simulink model "rfsoc4x2_ospfb_128"  (R2021a)
settings: Solver=VariableStepAuto  StartTime=0.0  StopTime=2048  RelTol=1e-3
undefined symbols (not defined in the file): pfb_coeff_gen_calc
libraries: xbsIndex_r4 x25898, casper_library_delays x113, casper_library_misc x68, xps_library x1
(part 146 of 221)

== system rfsoc4x2_ospfb_128/fft1/fft_direct/butterfly1_0/twiddle/bus_mult/mult1 ==
  a : Inport
  b : Inport  Port=2
  a_expand : Subsystem  AncestorBlock=casper_library_flow_control/bus_expand  mask(bus_expand){mode=divisions of equal size, outputNum=4, outputWidth=[18 18 18 18], outputBinaryPt=[17 17 17 17], outputArithmeticType=[1 1 1 1], show_format=off, outputToWorkspace=off, variablePrefix=out, outputToModelAsWell=on}
      mask prompts: outputNum "Number of outputs:"; outputWidth "Output width:"; outputBinaryPt "Output binary point position:"; outputArithmeticType "Output arithmetic type (ufix=0, fix=1, bool=2):"; show_format "Print format string?"; outputToWorkspace "Output to workspace?"; variablePrefix "Variable name prefix:"; outputToModelAsWell "Output to model as well?"
      mask help:
      | Expands a 'bus' made using a bus_create or Xilinx
      | concat block.
      | The input will be divided into the specified number
      | of outputs with the specified arithmetic types.
      | Divisions are made from most significant bit.
      mask init: same as rfsoc4x2_ospfb_128/bus_expand
      settings: AttributesFormatString=4 outputs
      mask TypeOptions mode: divisions of equal size | divisions of arbitrary size
      mask Callback mode: %bus_expand_callback();
      mask Callback outputWidth: %bus_expand_callback();
      mask Callback outputToWorkspace: %bus_expand_callback();
  a_replicate : Subsystem  AncestorBlock=casper_library_bus/bus_replicate  mask(bus_replicate){replication=2, csp_latency=0, misc=off, implementation=core}
      mask prompts: replication "replication factor"; csp_latency "latency"; misc "misc support"; implementation "delay implementation"
      mask help: Output bus formed by replicating input bus a number of times
      mask init:
      | bus_replicate_init(gcb, ...
      |     'replication', replication, ...
      |     'csp_latency', csp_latency, ...
      |     'implementation', implementation, ...
      |     'misc', misc);
      mask TypeOptions implementation: core | behavioral
  addsub_im : xbsIndex_r4/AddSub  mode=Addition  use_carryin=off  use_carryout=off  en=off  latency=2  precision=Full  arith_type=Unsigned  n_bits=16  bin_pt=14  quantization=Truncate  overflow=Wrap  use_behavioral_HDL=on  hw_selection=Fabric  pipelined=on  use_rpm=on  dbl_ovrd=off  block_type=addsub
  addsub_re : xbsIndex_r4/AddSub  mode=Subtraction  use_carryin=off  use_carryout=off  en=off  latency=2  precision=Full  arith_type=Unsigned  n_bits=16  bin_pt=14  quantization=Truncate  overflow=Wrap  use_behavioral_HDL=on  hw_selection=Fabric  pipelined=on  use_rpm=on  dbl_ovrd=off  block_type=addsub
  b_expand : Subsystem  AncestorBlock=casper_library_flow_control/bus_expand  mask(bus_expand){mode=divisions of equal size, outputNum=4, outputWidth=[18 18 18 18], outputBinaryPt=[17 17 17 17], outputArithmeticType=[1 1 1 1], show_format=off, outputToWorkspace=off, variablePrefix=out, outputToModelAsWell=on}
      mask prompts: outputNum "Number of outputs:"; outputWidth "Output width:"; outputBinaryPt "Output binary point position:"; outputArithmeticType "Output arithmetic type (ufix=0, fix=1, bool=2):"; show_format "Print format string?"; outputToWorkspace "Output to workspace?"; variablePrefix "Variable name prefix:"; outputToModelAsWell "Output to model as well?"
      mask help:
      | Expands a 'bus' made using a bus_create or Xilinx
      | concat block.
      | The input will be divided into the specified number
      | of outputs with the specified arithmetic types.
      | Divisions are made from most significant bit.
      mask init: same as rfsoc4x2_ospfb_128/bus_expand
      settings: AttributesFormatString=4 outputs
      mask TypeOptions mode: divisions of equal size | divisions of arbitrary size
      mask Callback mode: %bus_expand_callback();
      mask Callback outputWidth: %bus_expand_callback();
      mask Callback outputToWorkspace: %bus_expand_callback();
  b_replicate : Subsystem  AncestorBlock=casper_library_bus/bus_replicate  mask(bus_replicate){replication=2, csp_latency=0, misc=off, implementation=core}
      mask prompts: replication "replication factor"; csp_latency "latency"; misc "misc support"; implementation "delay implementation"
      mask help: Output bus formed by replicating input bus a number of times
      mask init:
      | bus_replicate_init(gcb, ...
      |     'replication', replication, ...
      |     'csp_latency', csp_latency, ...
      |     'implementation', implementation, ...
      |     'misc', misc);
      mask TypeOptions implementation: core | behavioral
  convert_im : xbsIndex_r4/Convert  gui_display_data_type=Fixed-point  arith_type="Signed  (2's comp)"  n_bits=37  bin_pt=34  float_type=Single  exp_bits=8  fraction_bits=24  quantization=Truncate  overflow=Wrap  en=off  latency=0  pipeline=on  dbl_ovrd=off  block_type=convert
  convert_re : xbsIndex_r4/Convert  gui_display_data_type=Fixed-point  arith_type="Signed  (2's comp)"  n_bits=37  bin_pt=34  float_type=Single  exp_bits=8  fraction_bits=24  quantization=Truncate  overflow=Wrap  en=off  latency=0  pipeline=on  dbl_ovrd=off  block_type=convert
  imim : xbsIndex_r4/Mult  precision=Full  arith_type="Signed  (2's comp)"  n_bits=16  bin_pt=14  quantization=Truncate  overflow=Wrap  en=off  latency=2  use_behavioral_HDL=on  opt=Speed  use_embedded=off  optimum_pipeline=off  pipeline=on  dbl_ovrd=off  use_rpm=on  placement_style=Triangular  block_type=mult
  imre : xbsIndex_r4/Mult  precision=Full  arith_type="Signed  (2's comp)"  n_bits=16  bin_pt=14  quantization=Truncate  overflow=Wrap  en=off  latency=2  use_behavioral_HDL=on  opt=Speed  use_embedded=off  optimum_pipeline=off  pipeline=on  dbl_ovrd=off  use_rpm=on  placement_style=Triangular  block_type=mult
  reim : xbsIndex_r4/Mult  precision=Full  arith_type="Signed  (2's comp)"  n_bits=16  bin_pt=14  quantization=Truncate  overflow=Wrap  en=off  latency=2  use_behavioral_HDL=on  opt=Speed  use_embedded=off  optimum_pipeline=off  pipeline=on  dbl_ovrd=off  use_rpm=on  placement_style=Triangular  block_type=mult
  rere : xbsIndex_r4/Mult  precision=Full  arith_type="Signed  (2's comp)"  n_bits=16  bin_pt=14  quantization=Truncate  overflow=Wrap  en=off  latency=2  use_behavioral_HDL=on  opt=Speed  use_embedded=off  optimum_pipeline=off  pipeline=on  dbl_ovrd=off  use_rpm=on  placement_style=Triangular  block_type=mult
  ri_to_c : Subsystem  AncestorBlock=casper_library_misc/ri_to_c  mask(ri_to_c){}
      mask help:
      | Concatenates real and imaginary inputs into a complex output.
      | Useful for simplifying interconnects.
      | See also: Complex to Real-Imag (c_to_ri)
      mask Help: eval('xlWeb(''http://casper.berkeley.edu/wiki/Ri_to_c'')')
  ab : Outport
  wires:
  a/1 -> a_replicate/1(in)
  b/1 -> b_replicate/1(in)
  a_replicate/1(out) -> a_expand/1(bus_in)
  b_replicate/1(out) -> b_expand/1(bus_in)
  a_expand/1(msb_out4) -> rere/1
  b_expand/1(msb_out4) -> rere/2
  a_expand/2(out3) -> imim/1
  b_expand/2(out3) -> imim/2
  a_expand/4(lsb_out1) -> imre/1
  b_expand/3(out2) -> imre/2
  a_expand/3(out2) -> reim/1
  b_expand/4(lsb_out1) -> reim/2
  rere/1 -> addsub_re/1
  imim/1 -> addsub_re/2
  imre/1 -> addsub_im/1
  reim/1 -> addsub_im/2
  addsub_re/1 -> convert_re/1
  addsub_im/1 -> convert_im/1
  convert_re/1 -> ri_to_c/1(re)
  convert_im/1 -> ri_to_c/2(im)
  ri_to_c/1(c) -> ab/1

== system rfsoc4x2_ospfb_128/fft1/fft_direct/butterfly1_0/twiddle/bus_mult/mult2 ==
  a : Inport
  b : Inport  Port=2
  a_expand : Subsystem  AncestorBlock=casper_library_flow_control/bus_expand  mask(bus_expand){mode=divisions of equal size, outputNum=4, outputWidth=[18 18 18 18], outputBinaryPt=[17 17 17 17], outputArithmeticType=[1 1 1 1], show_format=off, outputToWorkspace=off, variablePrefix=out, outputToModelAsWell=on}
      mask prompts: outputNum "Number of outputs:"; outputWidth "Output width:"; outputBinaryPt "Output binary point position:"; outputArithmeticType "Output arithmetic type (ufix=0, fix=1, bool=2):"; show_format "Print format string?"; outputToWorkspace "Output to workspace?"; variablePrefix "Variable name prefix:"; outputToModelAsWell "Output to model as well?"
      mask help:
      | Expands a 'bus' made using a bus_create or Xilinx
      | concat block.
      | The input will be divided into the specified number
      | of outputs with the specified arithmetic types.
      | Divisions are made from most significant bit.
      mask init: same as rfsoc4x2_ospfb_128/bus_expand
      settings: AttributesFormatString=4 outputs
      mask TypeOptions mode: divisions of equal size | divisions of arbitrary size
      mask Callback mode: %bus_expand_callback();
      mask Callback outputWidth: %bus_expand_callback();
      mask Callback outputToWorkspace: %bus_expand_callback();
  a_replicate : Subsystem  AncestorBlock=casper_library_bus/bus_replicate  mask(bus_replicate){replication=2, csp_latency=0, misc=off, implementation=core}
      mask prompts: replication "replication factor"; csp_latency "latency"; misc "misc support"; implementation "delay implementation"
      mask help: Output bus formed by replicating input bus a number of times
      mask init:
      | bus_replicate_init(gcb, ...
      |     'replication', replication, ...
      |     'csp_latency', csp_latency, ...
      |     'implementation', implementation, ...
      |     'misc', misc);
      mask TypeOptions implementation: core | behavioral
  addsub_im : xbsIndex_r4/AddSub  mode=Addition  use_carryin=off  use_carryout=off  en=off  latency=2  precision=Full  arith_type=Unsigned  n_bits=16  bin_pt=14  quantization=Truncate  overflow=Wrap  use_behavioral_HDL=on  hw_selection=Fabric  pipelined=on  use_rpm=on  dbl_ovrd=off  block_type=addsub
  addsub_re : xbsIndex_r4/AddSub  mode=Subtraction  use_carryin=off  use_carryout=off  en=off  latency=2  precision=Full  arith_type=Unsigned  n_bits=16  bin_pt=14  quantization=Truncate  overflow=Wrap  use_behavioral_HDL=on  hw_selection=Fabric  pipelined=on  use_rpm=on  dbl_ovrd=off  block_type=addsub
  b_expand : Subsystem  AncestorBlock=casper_library_flow_control/bus_expand  mask(bus_expand){mode=divisions of equal size, outputNum=4, outputWidth=[18 18 18 18], outputBinaryPt=[17 17 17 17], outputArithmeticType=[1 1 1 1], show_format=off, outputToWorkspace=off, variablePrefix=out, outputToModelAsWell=on}
      mask prompts: outputNum "Number of outputs:"; outputWidth "Output width:"; outputBinaryPt "Output binary point position:"; outputArithmeticType "Output arithmetic type (ufix=0, fix=1, bool=2):"; show_format "Print format string?"; outputToWorkspace "Output to workspace?"; variablePrefix "Variable name prefix:"; outputToModelAsWell "Output to model as well?"
      mask help:
      | Expands a 'bus' made using a bus_create or Xilinx
      | concat block.
      | The input will be divided into the specified number
      | of outputs with the specified arithmetic types.
      | Divisions are made from most significant bit.
      mask init: same as rfsoc4x2_ospfb_128/bus_expand
      settings: AttributesFormatString=4 outputs
      mask TypeOptions mode: divisions of equal size | divisions of arbitrary size
      mask Callback mode: %bus_expand_callback();
      mask Callback outputWidth: %bus_expand_callback();
      mask Callback outputToWorkspace: %bus_expand_callback();
  b_replicate : Subsystem  AncestorBlock=casper_library_bus/bus_replicate  mask(bus_replicate){replication=2, csp_latency=0, misc=off, implementation=core}
      mask prompts: replication "replication factor"; csp_latency "latency"; misc "misc support"; implementation "delay implementation"
      mask help: Output bus formed by replicating input bus a number of times
      mask init:
      | bus_replicate_init(gcb, ...
      |     'replication', replication, ...
      |     'csp_latency', csp_latency, ...
      |     'implementation', implementation, ...
      |     'misc', misc);
      mask TypeOptions implementation: core | behavioral
  convert_im : xbsIndex_r4/Convert  gui_display_data_type=Fixed-point  arith_type="Signed  (2's comp)"  n_bits=37  bin_pt=34  float_type=Single  exp_bits=8  fraction_bits=24  quantization=Truncate  overflow=Wrap  en=off  latency=0  pipeline=on  dbl_ovrd=off  block_type=convert
  convert_re : xbsIndex_r4/Convert  gui_display_data_type=Fixed-point  arith_type="Signed  (2's comp)"  n_bits=37  bin_pt=34  float_type=Single  exp_bits=8  fraction_bits=24  quantization=Truncate  overflow=Wrap  en=off  latency=0  pipeline=on  dbl_ovrd=off  block_type=convert
  imim : xbsIndex_r4/Mult  precision=Full  arith_type="Signed  (2's comp)"  n_bits=16  bin_pt=14  quantization=Truncate  overflow=Wrap  en=off  latency=2  use_behavioral_HDL=on  opt=Speed  use_embedded=off  optimum_pipeline=off  pipeline=on  dbl_ovrd=off  use_rpm=on  placement_style=Triangular  block_type=mult
  imre : xbsIndex_r4/Mult  precision=Full  arith_type="Signed  (2's comp)"  n_bits=16  bin_pt=14  quantization=Truncate  overflow=Wrap  en=off  latency=2  use_behavioral_HDL=on  opt=Speed  use_embedded=off  optimum_pipeline=off  pipeline=on  dbl_ovrd=off  use_rpm=on  placement_style=Triangular  block_type=mult
  reim : xbsIndex_r4/Mult  precision=Full  arith_type="Signed  (2's comp)"  n_bits=16  bin_pt=14  quantization=Truncate  overflow=Wrap  en=off  latency=2  use_behavioral_HDL=on  opt=Speed  use_embedded=off  optimum_pipeline=off  pipeline=on  dbl_ovrd=off  use_rpm=on  placement_style=Triangular  block_type=mult
  rere : xbsIndex_r4/Mult  precision=Full  arith_type="Signed  (2's comp)"  n_bits=16  bin_pt=14  quantization=Truncate  overflow=Wrap  en=off  latency=2  use_behavioral_HDL=on  opt=Speed  use_embedded=off  optimum_pipeline=off  pipeline=on  dbl_ovrd=off  use_rpm=on  placement_style=Triangular  block_type=mult
  ri_to_c : Subsystem  AncestorBlock=casper_library_misc/ri_to_c  mask(ri_to_c){}
      mask help:
      | Concatenates real and imaginary inputs into a complex output.
      | Useful for simplifying interconnects.
      | See also: Complex to Real-Imag (c_to_ri)
      mask Help: eval('xlWeb(''http://casper.berkeley.edu/wiki/Ri_to_c'')')
  ab : Outport
  wires:
  a/1 -> a_replicate/1(in)
  b/1 -> b_replicate/1(in)
  a_replicate/1(out) -> a_expand/1(bus_in)
  b_replicate/1(out) -> b_expand/1(bus_in)
  a_expand/1(msb_out4) -> rere/1
  b_expand/1(msb_out4) -> rere/2
  a_expand/2(out3) -> imim/1
  b_expand/2(out3) -> imim/2
  a_expand/4(lsb_out1) -> imre/1
  b_expand/3(out2) -> imre/2
  a_expand/3(out2) -> reim/1
  b_expand/4(lsb_out1) -> reim/2
  rere/1 -> addsub_re/1
  imim/1 -> addsub_re/2
  imre/1 -> addsub_im/1
  reim/1 -> addsub_im/2
  addsub_re/1 -> convert_re/1
  addsub_im/1 -> convert_im/1
  convert_re/1 -> ri_to_c/1(re)
  convert_im/1 -> ri_to_c/2(im)
  ri_to_c/1(c) -> ab/1

== system rfsoc4x2_ospfb_128/fft1/fft_direct/butterfly1_0/twiddle/bus_mult/repa ==
  in : Inport
  bussify : Subsystem  AncestorBlock=casper_library_flow_control/bus_create  mask(bus_create){inputNum=1}
      mask prompts: inputNum "Number of inputs:"
      mask init:
      | bus_create_init(gcb,...
      |     'inputNum', inputNum);
  out : Outport
  wires:
  in/1 -> bussify/1(in1)
  bussify/1(bus_out) -> out/1

== system rfsoc4x2_ospfb_128/fft1/fft_direct/butterfly1_0/twiddle/bus_mult/repb ==
  in : Inport
  bussify : Subsystem  AncestorBlock=casper_library_flow_control/bus_create  mask(bus_create){inputNum=1}
      mask prompts: inputNum "Number of inputs:"
      mask init:
      | bus_create_init(gcb,...
      |     'inputNum', inputNum);
  out : Outport
  wires:
  in/1 -> bussify/1(in1)
  bussify/1(bus_out) -> out/1

== system rfsoc4x2_ospfb_128/fft1/fft_direct/butterfly1_0/twiddle/coeff_gen/cosin ==
  theta : Inport
  misci : Inport  Port=2
  Constant4 : xbsIndex_r4/Constant  const=0  gui_display_data_type=Fixed-point  arith_type=Unsigned  n_bits=1  bin_pt=0  preci_type=Single  exp_width=8  frac_width=24  explicit_period=on  period=1  equ=P=C  opselect=C  inp2=PCIN>>17  opr=+  inp1=P  carry=CIN  dbl_ovrd=off  block_type=constant
  Constant5 : xbsIndex_r4/Constant  const=0  gui_display_data_type=Fixed-point  arith_type=Unsigned  n_bits=1  bin_pt=0  preci_type=Single  exp_width=8  frac_width=24  explicit_period=on  period=1  equ=P=C  opselect=C  inp2=PCIN>>17  opr=+  inp1=P  carry=CIN  dbl_ovrd=off  block_type=constant
  Delay : xbsIndex_r4/Delay  rst=off  infoeditControl=Selection of Reset will increase slice count due to use of real FFs and instead of SRLs  en=off  latency=bram_latency  reg_retiming=on  dbl_ovrd=off  block_type=delay
  Delay10 : xbsIndex_r4/Delay  rst=off  infoeditControl=Selection of Reset will increase slice count due to use of real FFs and instead of SRLs  en=off  latency=bram_latency  reg_retiming=on  dbl_ovrd=off  block_type=delay
  Delay8 : xbsIndex_r4/Delay  rst=off  infoeditControl=Selection of Reset will increase slice count due to use of real FFs and instead of SRLs  en=off  latency=bram_latency  reg_retiming=on  dbl_ovrd=off  block_type=delay
  ROM : xbsIndex_r4/ROM  depth=2^(6)  initVector=[34359476224 34349773679 34318575329 34266929750 34194574801 34101510483 33987998944 33854040184 33699634205 33525043154 33330267032 33115305841 32880421728 32625876837 32351409027 32057542588 31744539665 31412138116 31061124375 30691236301 30302736037 29896147875 29471471816 29029232149 28569166732 28092062000 27598180097 27087521024 26560609073 26017706387 25459075113 24885239541 24296199670 23692479791 23074866338 22443097167 21797696568 21139450974 20468098242 19784686950 19089479242 18382475119 17664461016 16935961220 16197237877 15448553131 14690955560 13924183021 13149021945 12365996623 11575631342 10778188247 9974191628 9164427916 8348897112 7528385649 6703417815 5874255754 5041685899 4206232538 3367895671 2527723875 1685979294 843448359]  distributed_mem=Block RAM  rst=off  init_reg=0  en=off  latency=bram_latency  gui_display_data_type=Fixed-point  arith_type=Unsigned  n_bits=n_bits*2  bin_pt=0  preci_type=Single  exp_width=8  frac_width=24  optimize=Speed  use_rpm=on  dbl_ovrd=off  simulation_type=fast_sim  block_type=sprom
  Terminator : Terminator
  Terminator1 : Terminator
  Terminator4 : Terminator
  add_convert0 : Subsystem
  add_convert1 : Subsystem
  assert : xbsIndex_r4/Assert  assert_type=on  type_source=Explicitly  gui_display_data_type=Fixed-point  arith_type=Unsigned  n_bits=6  bin_pt=0  preci_type=Single  exp_width=8  frac_width=24  assert_rate=off  rate_source=Explicitly  period=1  output_port=on  block_type=assert
  c_to_ri : casper_library_misc/c_to_ri  n_bits=n_bits  bin_pt=bin_pt
      settings: SourceProductName=CASPER DSP Blockset
  invert0 : Subsystem  mask{n_bits=n_bits, bin_pt=bin_pt, neg_latency=neg_latency, mux_latency=mux_latency}
      mask prompts: n_bits "bit width"; bin_pt "binary point"; neg_latency "negate latency"; mux_latency "mux latency"
  invert1 : Subsystem  mask{n_bits=n_bits, bin_pt=bin_pt, neg_latency=neg_latency, mux_latency=mux_latency}
      mask prompts: n_bits "bit width"; bin_pt "binary point"; neg_latency "negate latency"; mux_latency "mux latency"
  cos : Outport
  -sin : Outport  Port=2
  misco : Outport  Port=3
  wires:
  theta/1 -> assert/1
  assert/1 -> add_convert0/1(theta), add_convert1/1(theta)
  Constant4/1 -> add_convert0/2(misci)
  add_convert0/3(misco) -> Terminator/1
  misci/1 -> add_convert1/2(misci)
  add_convert1/3(misco) -> Delay/1
  add_convert0/2(add) -> ROM/1
  add_convert1/2(add) -> Terminator4/1
  ROM/1 -> c_to_ri/1
  add_convert1/1(negate) -> Delay8/1
  add_convert0/1(negate) -> Delay10/1
  Delay10/1 -> invert0/1(negate)
  Constant5/1 -> invert0/3(misci)
  c_to_ri/1 -> invert0/2(in)
  Delay8/1 -> invert1/1(negate)
  c_to_ri/2 -> invert1/2(in)
  invert0/2(misco) -> Terminator1/1
  Delay/1 -> invert1/3(misci)
  invert0/1(out) -> cos/1
  invert1/1(out) -> -sin/1
  invert1/2(misco) -> misco/1

== system rfsoc4x2_ospfb_128/fft1/fft_direct/butterfly1_1/twiddle/bus_convert/bussify ==
  in1 : Inport
  in2 : Inport  Port=2
  in3 : Inport  Port=3
  in4 : Inport  Port=4
  concatenate : xbsIndex_r4/Concat  num_inputs=4  dbl_ovrd=off  block_type=concat
  reinterpret{1..4} (4 alike) : xbsIndex_r4/Reinterpret  force_arith_type=on  arith_type=Unsigned  force_bin_pt=on  bin_pt=0  block_type=reinterpret
      reinterpret1 settings: infoedit="Changes signal type without altering the binary representation.   You can changed the signal between signed and unsigned, and relocate the binary point.<br><br>Hardware notes: In hardware this block costs nothing.<br><br>Example:  Suppose the input is 6 bits wide, signed, with 2 fractional bits, and the output is forced to unsigned with 0 fractional bits.  Then an input of -2.0 (1110.00 in binary 2's complement) becomes an output of 56 (111000 in binary)."
      reinterpret2 settings: infoedit="Changes signal type without altering the binary representation.   You can changed the signal between signed and unsigned, and relocate the binary point.<br><br>Hardware notes: In hardware this block costs nothing.<br><br>Example:  Suppose the input is 6 bits wide, signed, with 2 fractional bits, and the output is forced to unsigned with 0 fractional bits.  Then an input of -2.0 (1110.00 in binary 2's complement) becomes an output of 56 (111000 in binary)."
  bus_out : Outport  VectorParamsAs1DForOutWhenUnconnected=off
  wires:
  concatenate/1 -> bus_out/1
  in1/1 -> reinterpret1/1
  reinterpret1/1 -> concatenate/1
  in2/1 -> reinterpret2/1
  reinterpret2/1 -> concatenate/2
  in3/1 -> reinterpret3/1
  reinterpret3/1 -> concatenate/3
  in4/1 -> reinterpret4/1
  reinterpret4/1 -> concatenate/4

== system rfsoc4x2_ospfb_128/fft1/fft_direct/butterfly1_1/twiddle/bus_convert/debus ==
  bus_in : Inport
  reinterpret{1..4} (4 alike) : xbsIndex_r4/Reinterpret  force_arith_type=on  arith_type="Signed  (2's comp)"  force_bin_pt=on  bin_pt=34  block_type=reinterpret
  slice1 : xbsIndex_r4/Slice  nbits=37  boolean_output=off  mode=Upper Bit Location + Width  bit1=-111  base1=MSB of Input  bit0=0  base0=LSB of Input  dbl_ovrd=off  block_type=slice
  slice2 : xbsIndex_r4/Slice  nbits=37  boolean_output=off  mode=Upper Bit Location + Width  bit1=-74  base1=MSB of Input  bit0=0  base0=LSB of Input  dbl_ovrd=off  block_type=slice
  slice3 : xbsIndex_r4/Slice  nbits=37  boolean_output=off  mode=Upper Bit Location + Width  bit1=-37  base1=MSB of Input  bit0=0  base0=LSB of Input  dbl_ovrd=off  block_type=slice
  slice4 : xbsIndex_r4/Slice  nbits=37  boolean_output=off  mode=Upper Bit Location + Width  bit1=0  base1=MSB of Input  bit0=0  base0=LSB of Input  dbl_ovrd=off  block_type=slice
  msb_out4 : Outport
  out3 : Outport  Port=2
  out2 : Outport  Port=3
  lsb_out1 : Outport  Port=4  VectorParamsAs1DForOutWhenUnconnected=off
  wires:
  bus_in/1 -> slice4/1, slice3/1, slice2/1, slice1/1
  slice4/1 -> reinterpret4/1
  reinterpret4/1 -> msb_out4/1
  slice3/1 -> reinterpret3/1
  reinterpret3/1 -> out3/1
  slice2/1 -> reinterpret2/1
  reinterpret2/1 -> out2/1
  slice1/1 -> reinterpret1/1
  reinterpret1/1 -> lsb_out1/1

== system rfsoc4x2_ospfb_128/fft1/fft_direct/butterfly1_1/twiddle/bus_mult/a*b_bussify ==
  in1 : Inport
  in2 : Inport  Port=2
  concatenate : xbsIndex_r4/Concat  num_inputs=2  dbl_ovrd=off  block_type=concat
  reinterpret1 : xbsIndex_r4/Reinterpret  force_arith_type=on  arith_type=Unsigned  force_bin_pt=on  bin_pt=0  block_type=reinterpret
      settings: infoedit="Changes signal type without altering the binary representation.   You can changed the signal between signed and unsigned, and relocate the binary point.<br><br>Hardware notes: In hardware this block costs nothing.<br><br>Example:  Suppose the input is 6 bits wide, signed, with 2 fractional bits, and the output is forced to unsigned with 0 fractional bits.  Then an input of -2.0 (1110.00 in binary 2's complement) becomes an output of 56 (111000 in binary)."
  reinterpret2 : xbsIndex_r4/Reinterpret  force_arith_type=on  arith_type=Unsigned  force_bin_pt=on  bin_pt=0  block_type=reinterpret
  bus_out : Outport  VectorParamsAs1DForOutWhenUnconnected=off
  wires:
  concatenate/1 -> bus_out/1
  in1/1 -> reinterpret1/1
  reinterpret1/1 -> concatenate/1
  in2/1 -> reinterpret2/1
  reinterpret2/1 -> concatenate/2

== system rfsoc4x2_ospfb_128/fft1/fft_direct/butterfly1_1/twiddle/bus_mult/a_debus ==
  bus_in : Inport
  reinterpret1 : xbsIndex_r4/Reinterpret  force_arith_type=on  arith_type=Unsigned  force_bin_pt=on  bin_pt=0  block_type=reinterpret
  slice1 : xbsIndex_r4/Slice  nbits=36  boolean_output=off  mode=Upper Bit Location + Width  bit1=0  base1=MSB of Input  bit0=0  base0=LSB of Input  dbl_ovrd=off  block_type=slice
  msb_lsb_out1 : Outport
  wires:
  bus_in/1 -> slice1/1
  slice1/1 -> reinterpret1/1
  reinterpret1/1 -> msb_lsb_out1/1

== system rfsoc4x2_ospfb_128/fft1/fft_direct/butterfly1_1/twiddle/bus_mult/b_debus ==
  bus_in : Inport
  reinterpret1 : xbsIndex_r4/Reinterpret  force_arith_type=on  arith_type=Unsigned  force_bin_pt=on  bin_pt=0  block_type=reinterpret
  reinterpret2 : xbsIndex_r4/Reinterpret  force_arith_type=on  arith_type=Unsigned  force_bin_pt=on  bin_pt=0  block_type=reinterpret
  slice1 : xbsIndex_r4/Slice  nbits=36  boolean_output=off  mode=Upper Bit Location + Width  bit1=-36  base1=MSB of Input  bit0=0  base0=LSB of Input  dbl_ovrd=off  block_type=slice
  slice2 : xbsIndex_r4/Slice  nbits=36  boolean_output=off  mode=Upper Bit Location + Width  bit1=0  base1=MSB of Input  bit0=0  base0=LSB of Input  dbl_ovrd=off  block_type=slice
  msb_out2 : Outport
  lsb_out1 : Outport  Port=2
  wires:
  bus_in/1 -> slice2/1, slice1/1
  slice2/1 -> reinterpret2/1
  reinterpret2/1 -> msb_out2/1
  slice1/1 -> reinterpret1/1
  reinterpret1/1 -> lsb_out1/1

== system rfsoc4x2_ospfb_128/fft1/fft_direct/butterfly1_1/twiddle/bus_mult/mult1 ==
  a : Inport
  b : Inport  Port=2
  a_expand : Subsystem  AncestorBlock=casper_library_flow_control/bus_expand  mask(bus_expand){mode=divisions of equal size, outputNum=4, outputWidth=[18 18 18 18], outputBinaryPt=[17 17 17 17], outputArithmeticType=[1 1 1 1], show_format=off, outputToWorkspace=off, variablePrefix=out, outputToModelAsWell=on}
      mask prompts: outputNum "Number of outputs:"; outputWidth "Output width:"; outputBinaryPt "Output binary point position:"; outputArithmeticType "Output arithmetic type (ufix=0, fix=1, bool=2):"; show_format "Print format string?"; outputToWorkspace "Output to workspace?"; variablePrefix "Variable name prefix:"; outputToModelAsWell "Output to model as well?"
      mask help:
      | Expands a 'bus' made using a bus_create or Xilinx
      | concat block.
      | The input will be divided into the specified number
      | of outputs with the specified arithmetic types.
      | Divisions are made from most significant bit.
      mask init: same as rfsoc4x2_ospfb_128/bus_expand
      settings: AttributesFormatString=4 outputs
      mask TypeOptions mode: divisions of equal size | divisions of arbitrary size
      mask Callback mode: %bus_expand_callback();
      mask Callback outputWidth: %bus_expand_callback();
      mask Callback outputToWorkspace: %bus_expand_callback();
  a_replicate : Subsystem  AncestorBlock=casper_library_bus/bus_replicate  mask(bus_replicate){replication=2, csp_latency=0, misc=off, implementation=core}
      mask prompts: replication "replication factor"; csp_latency "latency"; misc "misc support"; implementation "delay implementation"
      mask help: Output bus formed by replicating input bus a number of times
      mask init:
      | bus_replicate_init(gcb, ...
      |     'replication', replication, ...
      |     'csp_latency', csp_latency, ...
      |     'implementation', implementation, ...
      |     'misc', misc);
      mask TypeOptions implementation: core | behavioral
  addsub_im : xbsIndex_r4/AddSub  mode=Addition  use_carryin=off  use_carryout=off  en=off  latency=2  precision=Full  arith_type=Unsigned  n_bits=16  bin_pt=14  quantization=Truncate  overflow=Wrap  use_behavioral_HDL=on  hw_selection=Fabric  pipelined=on  use_rpm=on  dbl_ovrd=off  block_type=addsub
  addsub_re : xbsIndex_r4/AddSub  mode=Subtraction  use_carryin=off  use_carryout=off  en=off  latency=2  precision=Full  arith_type=Unsigned  n_bits=16  bin_pt=14  quantization=Truncate  overflow=Wrap  use_behavioral_HDL=on  hw_selection=Fabric  pipelined=on  use_rpm=on  dbl_ovrd=off  block_type=addsub
  b_expand : Subsystem  AncestorBlock=casper_library_flow_control/bus_expand  mask(bus_expand){mode=divisions of equal size, outputNum=4, outputWidth=[18 18 18 18], outputBinaryPt=[17 17 17 17], outputArithmeticType=[1 1 1 1], show_format=off, outputToWorkspace=off, variablePrefix=out, outputToModelAsWell=on}
      mask prompts: outputNum "Number of outputs:"; outputWidth "Output width:"; outputBinaryPt "Output binary point position:"; outputArithmeticType "Output arithmetic type (ufix=0, fix=1, bool=2):"; show_format "Print format string?"; outputToWorkspace "Output to workspace?"; variablePrefix "Variable name prefix:"; outputToModelAsWell "Output to model as well?"
      mask help:
      | Expands a 'bus' made using a bus_create or Xilinx
      | concat block.
      | The input will be divided into the specified number
      | of outputs with the specified arithmetic types.
      | Divisions are made from most significant bit.
      mask init: same as rfsoc4x2_ospfb_128/bus_expand
      settings: AttributesFormatString=4 outputs
      mask TypeOptions mode: divisions of equal size | divisions of arbitrary size
      mask Callback mode: %bus_expand_callback();
      mask Callback outputWidth: %bus_expand_callback();
      mask Callback outputToWorkspace: %bus_expand_callback();
  b_replicate : Subsystem  AncestorBlock=casper_library_bus/bus_replicate  mask(bus_replicate){replication=2, csp_latency=0, misc=off, implementation=core}
      mask prompts: replication "replication factor"; csp_latency "latency"; misc "misc support"; implementation "delay implementation"
      mask help: Output bus formed by replicating input bus a number of times
      mask init:
      | bus_replicate_init(gcb, ...
      |     'replication', replication, ...
      |     'csp_latency', csp_latency, ...
      |     'implementation', implementation, ...
      |     'misc', misc);
      mask TypeOptions implementation: core | behavioral
  convert_im : xbsIndex_r4/Convert  gui_display_data_type=Fixed-point  arith_type="Signed  (2's comp)"  n_bits=37  bin_pt=34  float_type=Single  exp_bits=8  fraction_bits=24  quantization=Truncate  overflow=Wrap  en=off  latency=0  pipeline=on  dbl_ovrd=off  block_type=convert
  convert_re : xbsIndex_r4/Convert  gui_display_data_type=Fixed-point  arith_type="Signed  (2's comp)"  n_bits=37  bin_pt=34  float_type=Single  exp_bits=8  fraction_bits=24  quantization=Truncate  overflow=Wrap  en=off  latency=0  pipeline=on  dbl_ovrd=off  block_type=convert
  imim : xbsIndex_r4/Mult  precision=Full  arith_type="Signed  (2's comp)"  n_bits=16  bin_pt=14  quantization=Truncate  overflow=Wrap  en=off  latency=2  use_behavioral_HDL=on  opt=Speed  use_embedded=off  optimum_pipeline=off  pipeline=on  dbl_ovrd=off  use_rpm=on  placement_style=Triangular  block_type=mult
  imre : xbsIndex_r4/Mult  precision=Full  arith_type="Signed  (2's comp)"  n_bits=16  bin_pt=14  quantization=Truncate  overflow=Wrap  en=off  latency=2  use_behavioral_HDL=on  opt=Speed  use_embedded=off  optimum_pipeline=off  pipeline=on  dbl_ovrd=off  use_rpm=on  placement_style=Triangular  block_type=mult
  reim : xbsIndex_r4/Mult  precision=Full  arith_type="Signed  (2's comp)"  n_bits=16  bin_pt=14  quantization=Truncate  overflow=Wrap  en=off  latency=2  use_behavioral_HDL=on  opt=Speed  use_embedded=off  optimum_pipeline=off  pipeline=on  dbl_ovrd=off  use_rpm=on  placement_style=Triangular  block_type=mult
  rere : xbsIndex_r4/Mult  precision=Full  arith_type="Signed  (2's comp)"  n_bits=16  bin_pt=14  quantization=Truncate  overflow=Wrap  en=off  latency=2  use_behavioral_HDL=on  opt=Speed  use_embedded=off  optimum_pipeline=off  pipeline=on  dbl_ovrd=off  use_rpm=on  placement_style=Triangular  block_type=mult
  ri_to_c : Subsystem  AncestorBlock=casper_library_misc/ri_to_c  mask(ri_to_c){}
      mask help:
      | Concatenates real and imaginary inputs into a complex output.
      | Useful for simplifying interconnects.
      | See also: Complex to Real-Imag (c_to_ri)
      mask Help: eval('xlWeb(''http://casper.berkeley.edu/wiki/Ri_to_c'')')
  ab : Outport
  wires:
  a/1 -> a_replicate/1(in)
  b/1 -> b_replicate/1(in)
  a_replicate/1(out) -> a_expand/1(bus_in)
  b_replicate/1(out) -> b_expand/1(bus_in)
  a_expand/1(msb_out4) -> rere/1
  b_expand/1(msb_out4) -> rere/2
  a_expand/2(out3) -> imim/1
  b_expand/2(out3) -> imim/2
  a_expand/4(lsb_out1) -> imre/1
  b_expand/3(out2) -> imre/2
  a_expand/3(out2) -> reim/1
  b_expand/4(lsb_out1) -> reim/2
  rere/1 -> addsub_re/1
  imim/1 -> addsub_re/2
  imre/1 -> addsub_im/1
  reim/1 -> addsub_im/2
  addsub_re/1 -> convert_re/1
  addsub_im/1 -> convert_im/1
  convert_re/1 -> ri_to_c/1(re)
  convert_im/1 -> ri_to_c/2(im)
  ri_to_c/1(c) -> ab/1

== system rfsoc4x2_ospfb_128/fft1/fft_direct/butterfly1_1/twiddle/bus_mult/mult2 ==
  a : Inport
  b : Inport  Port=2
  a_expand : Subsystem  AncestorBlock=casper_library_flow_control/bus_expand  mask(bus_expand){mode=divisions of equal size, outputNum=4, outputWidth=[18 18 18 18], outputBinaryPt=[17 17 17 17], outputArithmeticType=[1 1 1 1], show_format=off, outputToWorkspace=off, variablePrefix=out, outputToModelAsWell=on}
      mask prompts: outputNum "Number of outputs:"; outputWidth "Output width:"; outputBinaryPt "Output binary point position:"; outputArithmeticType "Output arithmetic type (ufix=0, fix=1, bool=2):"; show_format "Print format string?"; outputToWorkspace "Output to workspace?"; variablePrefix "Variable name prefix:"; outputToModelAsWell "Output to model as well?"
      mask help:
      | Expands a 'bus' made using a bus_create or Xilinx
      | concat block.
      | The input will be divided into the specified number
      | of outputs with the specified arithmetic types.
      | Divisions are made from most significant bit.
      mask init: same as rfsoc4x2_ospfb_128/bus_expand
      settings: AttributesFormatString=4 outputs
      mask TypeOptions mode: divisions of equal size | divisions of arbitrary size
      mask Callback mode: %bus_expand_callback();
      mask Callback outputWidth: %bus_expand_callback();
      mask Callback outputToWorkspace: %bus_expand_callback();
  a_replicate : Subsystem  AncestorBlock=casper_library_bus/bus_replicate  mask(bus_replicate){replication=2, csp_latency=0, misc=off, implementation=core}
      mask prompts: replication "replication factor"; csp_latency "latency"; misc "misc support"; implementation "delay implementation"
      mask help: Output bus formed by replicating input bus a number of times
      mask init:
      | bus_replicate_init(gcb, ...
      |     'replication', replication, ...
      |     'csp_latency', csp_latency, ...
      |     'implementation', implementation, ...
      |     'misc', misc);
      mask TypeOptions implementation: core | behavioral
  addsub_im : xbsIndex_r4/AddSub  mode=Addition  use_carryin=off  use_carryout=off  en=off  latency=2  precision=Full  arith_type=Unsigned  n_bits=16  bin_pt=14  quantization=Truncate  overflow=Wrap  use_behavioral_HDL=on  hw_selection=Fabric  pipelined=on  use_rpm=on  dbl_ovrd=off  block_type=addsub
  addsub_re : xbsIndex_r4/AddSub  mode=Subtraction  use_carryin=off  use_carryout=off  en=off  latency=2  precision=Full  arith_type=Unsigned  n_bits=16  bin_pt=14  quantization=Truncate  overflow=Wrap  use_behavioral_HDL=on  hw_selection=Fabric  pipelined=on  use_rpm=on  dbl_ovrd=off  block_type=addsub
  b_expand : Subsystem  AncestorBlock=casper_library_flow_control/bus_expand  mask(bus_expand){mode=divisions of equal size, outputNum=4, outputWidth=[18 18 18 18], outputBinaryPt=[17 17 17 17], outputArithmeticType=[1 1 1 1], show_format=off, outputToWorkspace=off, variablePrefix=out, outputToModelAsWell=on}
      mask prompts: outputNum "Number of outputs:"; outputWidth "Output width:"; outputBinaryPt "Output binary point position:"; outputArithmeticType "Output arithmetic type (ufix=0, fix=1, bool=2):"; show_format "Print format string?"; outputToWorkspace "Output to workspace?"; variablePrefix "Variable name prefix:"; outputToModelAsWell "Output to model as well?"
      mask help:
      | Expands a 'bus' made using a bus_create or Xilinx
      | concat block.
      | The input will be divided into the specified number
      | of outputs with the specified arithmetic types.
      | Divisions are made from most significant bit.
      mask init: same as rfsoc4x2_ospfb_128/bus_expand
      settings: AttributesFormatString=4 outputs
      mask TypeOptions mode: divisions of equal size | divisions of arbitrary size
      mask Callback mode: %bus_expand_callback();
      mask Callback outputWidth: %bus_expand_callback();
      mask Callback outputToWorkspace: %bus_expand_callback();
  b_replicate : Subsystem  AncestorBlock=casper_library_bus/bus_replicate  mask(bus_replicate){replication=2, csp_latency=0, misc=off, implementation=core}
      mask prompts: replication "replication factor"; csp_latency "latency"; misc "misc support"; implementation "delay implementation"
      mask help: Output bus formed by replicating input bus a number of times
      mask init:
      | bus_replicate_init(gcb, ...
      |     'replication', replication, ...
      |     'csp_latency', csp_latency, ...
      |     'implementation', implementation, ...
      |     'misc', misc);
      mask TypeOptions implementation: core | behavioral
  convert_im : xbsIndex_r4/Convert  gui_display_data_type=Fixed-point  arith_type="Signed  (2's comp)"  n_bits=37  bin_pt=34  float_type=Single  exp_bits=8  fraction_bits=24  quantization=Truncate  overflow=Wrap  en=off  latency=0  pipeline=on  dbl_ovrd=off  block_type=convert
  convert_re : xbsIndex_r4/Convert  gui_display_data_type=Fixed-point  arith_type="Signed  (2's comp)"  n_bits=37  bin_pt=34  float_type=Single  exp_bits=8  fraction_bits=24  quantization=Truncate  overflow=Wrap  en=off  latency=0  pipeline=on  dbl_ovrd=off  block_type=convert
  imim : xbsIndex_r4/Mult  precision=Full  arith_type="Signed  (2's comp)"  n_bits=16  bin_pt=14  quantization=Truncate  overflow=Wrap  en=off  latency=2  use_behavioral_HDL=on  opt=Speed  use_embedded=off  optimum_pipeline=off  pipeline=on  dbl_ovrd=off  use_rpm=on  placement_style=Triangular  block_type=mult
  imre : xbsIndex_r4/Mult  precision=Full  arith_type="Signed  (2's comp)"  n_bits=16  bin_pt=14  quantization=Truncate  overflow=Wrap  en=off  latency=2  use_behavioral_HDL=on  opt=Speed  use_embedded=off  optimum_pipeline=off  pipeline=on  dbl_ovrd=off  use_rpm=on  placement_style=Triangular  block_type=mult
  reim : xbsIndex_r4/Mult  precision=Full  arith_type="Signed  (2's comp)"  n_bits=16  bin_pt=14  quantization=Truncate  overflow=Wrap  en=off  latency=2  use_behavioral_HDL=on  opt=Speed  use_embedded=off  optimum_pipeline=off  pipeline=on  dbl_ovrd=off  use_rpm=on  placement_style=Triangular  block_type=mult
  rere : xbsIndex_r4/Mult  precision=Full  arith_type="Signed  (2's comp)"  n_bits=16  bin_pt=14  quantization=Truncate  overflow=Wrap  en=off  latency=2  use_behavioral_HDL=on  opt=Speed  use_embedded=off  optimum_pipeline=off  pipeline=on  dbl_ovrd=off  use_rpm=on  placement_style=Triangular  block_type=mult
  ri_to_c : Subsystem  AncestorBlock=casper_library_misc/ri_to_c  mask(ri_to_c){}
      mask help:
      | Concatenates real and imaginary inputs into a complex output.
      | Useful for simplifying interconnects.
      | See also: Complex to Real-Imag (c_to_ri)
      mask Help: eval('xlWeb(''http://casper.berkeley.edu/wiki/Ri_to_c'')')
  ab : Outport
  wires:
  a/1 -> a_replicate/1(in)
  b/1 -> b_replicate/1(in)
  a_replicate/1(out) -> a_expand/1(bus_in)
  b_replicate/1(out) -> b_expand/1(bus_in)
  a_expand/1(msb_out4) -> rere/1
  b_expand/1(msb_out4) -> rere/2
  a_expand/2(out3) -> imim/1
  b_expand/2(out3) -> imim/2
  a_expand/4(lsb_out1) -> imre/1
  b_expand/3(out2) -> imre/2
  a_expand/3(out2) -> reim/1
  b_expand/4(lsb_out1) -> reim/2
  rere/1 -> addsub_re/1
  imim/1 -> addsub_re/2
  imre/1 -> addsub_im/1
  reim/1 -> addsub_im/2
  addsub_re/1 -> convert_re/1
  addsub_im/1 -> convert_im/1
  convert_re/1 -> ri_to_c/1(re)
  convert_im/1 -> ri_to_c/2(im)
  ri_to_c/1(c) -> ab/1

== system rfsoc4x2_ospfb_128/fft1/fft_direct/butterfly1_1/twiddle/bus_mult/repa ==
  in : Inport
  bussify : Subsystem  AncestorBlock=casper_library_flow_control/bus_create  mask(bus_create){inputNum=1}
      mask prompts: inputNum "Number of inputs:"
      mask init:
      | bus_create_init(gcb,...
      |     'inputNum', inputNum);
  out : Outport
  wires:
  in/1 -> bussify/1(in1)
  bussify/1(bus_out) -> out/1

== system rfsoc4x2_ospfb_128/fft1/fft_direct/butterfly1_1/twiddle/bus_mult/repb ==
  in : Inport
  bussify : Subsystem  AncestorBlock=casper_library_flow_control/bus_create  mask(bus_create){inputNum=1}
      mask prompts: inputNum "Number of inputs:"
      mask init:
      | bus_create_init(gcb,...
      |     'inputNum', inputNum);
  out : Outport
  wires:
  in/1 -> bussify/1(in1)
  bussify/1(bus_out) -> out/1

== system rfsoc4x2_ospfb_128/fft1/fft_direct/butterfly1_1/twiddle/coeff_gen/cosin ==
  theta : Inport
  misci : Inport  Port=2
  Constant4 : xbsIndex_r4/Constant  const=0  gui_display_data_type=Fixed-point  arith_type=Unsigned  n_bits=1  bin_pt=0  preci_type=Single  exp_width=8  frac_width=24  explicit_period=on  period=1  equ=P=C  opselect=C  inp2=PCIN>>17  opr=+  inp1=P  carry=CIN  dbl_ovrd=off  block_type=constant
  Constant5 : xbsIndex_r4/Constant  const=0  gui_display_data_type=Fixed-point  arith_type=Unsigned  n_bits=1  bin_pt=0  preci_type=Single  exp_width=8  frac_width=24  explicit_period=on  period=1  equ=P=C  opselect=C  inp2=PCIN>>17  opr=+  inp1=P  carry=CIN  dbl_ovrd=off  block_type=constant
  Delay : xbsIndex_r4/Delay  rst=off  infoeditControl=Selection of Reset will increase slice count due to use of real FFs and instead of SRLs  en=off  latency=bram_latency  reg_retiming=on  dbl_ovrd=off  block_type=delay
  Delay10 : xbsIndex_r4/Delay  rst=off  infoeditControl=Selection of Reset will increase slice count due to use of real FFs and instead of SRLs  en=off  latency=bram_latency  reg_retiming=on  dbl_ovrd=off  block_type=delay
  Delay8 : xbsIndex_r4/Delay  rst=off  infoeditControl=Selection of Reset will increase slice count due to use of real FFs and instead of SRLs  en=off  latency=bram_latency  reg_retiming=on  dbl_ovrd=off  block_type=delay
  ROM : xbsIndex_r4/ROM  depth=2^(6)  initVector=[131072 67876290599 67033759902 66192015715 65351844471 64513508314 63678055819 62845486986 62016326103 61191359601 60370849624 59555320460 58745558540 57941563863 57144122862 56353759823 55570736889 54795578349 54028808488 53271213739 52522531957 51783811716 51055315160 50337304431 49630303818 48935099750 48251692226 47580343390 46922101816 46276705359 45644940450 45027331375 44423615990 43834580725 43260749865 42702123411 42159225649 41632318720 41121664769 40627788080 40150688652 39690628629 39248394440 38823723939 38417141413 38028646861 37658764567 37307756676 36975361041 36662364092 36368503683 36094041957 35839503200 35604625265 35389670296 35194900434 35020315677 34865916024 34731963616 34618458451 34525400529 34453051990 34401412833 34370220911]  distributed_mem=Block RAM  rst=off  init_reg=0  en=off  latency=bram_latency  gui_display_data_type=Fixed-point  arith_type=Unsigned  n_bits=n_bits*2  bin_pt=0  preci_type=Single  exp_width=8  frac_width=24  optimize=Speed  use_rpm=on  dbl_ovrd=off  simulation_type=fast_sim  block_type=sprom
  Terminator : Terminator
  Terminator1 : Terminator
  Terminator4 : Terminator
  add_convert0 : Subsystem
  add_convert1 : Subsystem
  assert : xbsIndex_r4/Assert  assert_type=on  type_source=Explicitly  gui_display_data_type=Fixed-point  arith_type=Unsigned  n_bits=6  bin_pt=0  preci_type=Single  exp_width=8  frac_width=24  assert_rate=off  rate_source=Explicitly  period=1  output_port=on  block_type=assert
  c_to_ri : casper_library_misc/c_to_ri  n_bits=n_bits  bin_pt=bin_pt
      settings: SourceProductName=CASPER DSP Blockset
  invert0 : Subsystem  mask{n_bits=n_bits, bin_pt=bin_pt, neg_latency=neg_latency, mux_latency=mux_latency}
      mask prompts: n_bits "bit width"; bin_pt "binary point"; neg_latency "negate latency"; mux_latency "mux latency"
  invert1 : Subsystem  mask{n_bits=n_bits, bin_pt=bin_pt, neg_latency=neg_latency, mux_latency=mux_latency}
      mask prompts: n_bits "bit width"; bin_pt "binary point"; neg_latency "negate latency"; mux_latency "mux latency"
  -sin : Outport
  -cos : Outport  Port=2
  misco : Outport  Port=3
  wires:
  theta/1 -> assert/1
  assert/1 -> add_convert0/1(theta), add_convert1/1(theta)
  Constant4/1 -> add_convert0/2(misci)
  add_convert0/3(misco) -> Terminator/1
  misci/1 -> add_convert1/2(misci)
  add_convert1/3(misco) -> Delay/1
  add_convert0/2(add) -> ROM/1
  add_convert1/2(add) -> Terminator4/1
  ROM/1 -> c_to_ri/1
  add_convert1/1(negate) -> Delay8/1
  add_convert0/1(negate) -> Delay10/1
  Delay10/1 -> invert0/1(negate)
  Constant5/1 -> invert0/3(misci)
  c_to_ri/1 -> invert0/2(in)
  Delay8/1 -> invert1/1(negate)
  c_to_ri/2 -> invert1/2(in)
  invert0/2(misco) -> Terminator1/1
  Delay/1 -> invert1/3(misci)
  invert0/1(out) -> -sin/1
  invert1/1(out) -> -cos/1
  invert1/2(misco) -> misco/1

== system rfsoc4x2_ospfb_128/fft1/fft_direct/butterfly2_0/twiddle/bus_convert/bussify ==
  in1 : Inport
  in2 : Inport  Port=2
  concatenate : xbsIndex_r4/Concat  num_inputs=2  dbl_ovrd=off  block_type=concat
  reinterpret1 : xbsIndex_r4/Reinterpret  force_arith_type=on  arith_type=Unsigned  force_bin_pt=on  bin_pt=0  block_type=reinterpret
      settings: infoedit="Changes signal type without altering the binary representation.   You can changed the signal between signed and unsigned, and relocate the binary point.<br><br>Hardware notes: In hardware this block costs nothing.<br><br>Example:  Suppose the input is 6 bits wide, signed, with 2 fractional bits, and the output is forced to unsigned with 0 fractional bits.  Then an input of -2.0 (1110.00 in binary 2's complement) becomes an output of 56 (111000 in binary)."
  reinterpret2 : xbsIndex_r4/Reinterpret  force_arith_type=on  arith_type=Unsigned  force_bin_pt=on  bin_pt=0  block_type=reinterpret
      settings: infoedit="Changes signal type without altering the binary representation.   You can changed the signal between signed and unsigned, and relocate the binary point.<br><br>Hardware notes: In hardware this block costs nothing.<br><br>Example:  Suppose the input is 6 bits wide, signed, with 2 fractional bits, and the output is forced to unsigned with 0 fractional bits.  Then an input of -2.0 (1110.00 in binary 2's complement) becomes an output of 56 (111000 in binary)."
  bus_out : Outport  VectorParamsAs1DForOutWhenUnconnected=off
  wires:
  concatenate/1 -> bus_out/1
  in1/1 -> reinterpret1/1
  reinterpret1/1 -> concatenate/1
  in2/1 -> reinterpret2/1
  reinterpret2/1 -> concatenate/2

== system rfsoc4x2_ospfb_128/fft1/fft_direct/butterfly2_0/twiddle/bus_convert/debus ==
  bus_in : Inport
  reinterpret1 : xbsIndex_r4/Reinterpret  force_arith_type=on  arith_type="Signed  (2's comp)"  force_bin_pt=on  bin_pt=34  block_type=reinterpret
  reinterpret2 : xbsIndex_r4/Reinterpret  force_arith_type=on  arith_type="Signed  (2's comp)"  force_bin_pt=on  bin_pt=34  block_type=reinterpret
  slice1 : xbsIndex_r4/Slice  nbits=37  boolean_output=off  mode=Upper Bit Location + Width  bit1=-37  base1=MSB of Input  bit0=0  base0=LSB of Input  dbl_ovrd=off  block_type=slice
  slice2 : xbsIndex_r4/Slice  nbits=37  boolean_output=off  mode=Upper Bit Location + Width  bit1=0  base1=MSB of Input  bit0=0  base0=LSB of Input  dbl_ovrd=off  block_type=slice
  msb_out2 : Outport  VectorParamsAs1DForOutWhenUnconnected=off
  lsb_out1 : Outport  Port=2  VectorParamsAs1DForOutWhenUnconnected=off
  wires:
  bus_in/1 -> slice2/1, slice1/1
  slice2/1 -> reinterpret2/1
  reinterpret2/1 -> msb_out2/1
  slice1/1 -> reinterpret1/1
  reinterpret1/1 -> lsb_out1/1

== system rfsoc4x2_ospfb_128/fft1/fft_direct/butterfly2_0/twiddle/bus_mult/a*b_bussify ==
  in1 : Inport
  reinterpret1 : xbsIndex_r4/Reinterpret  force_arith_type=on  arith_type=Unsigned  force_bin_pt=on  bin_pt=0  block_type=reinterpret
      settings: infoedit="Changes signal type without altering the binary representation.   You can changed the signal between signed and unsigned, and relocate the binary point.<br><br>Hardware notes: In hardware this block costs nothing.<br><br>Example:  Suppose the input is 6 bits wide, signed, with 2 fractional bits, and the output is forced to unsigned with 0 fractional bits.  Then an input of -2.0 (1110.00 in binary 2's complement) becomes an output of 56 (111000 in binary)."
  bus_out : Outport  VectorParamsAs1DForOutWhenUnconnected=off
  wires:
  in1/1 -> reinterpret1/1
  reinterpret1/1 -> bus_out/1

== system rfsoc4x2_ospfb_128/fft1/fft_direct/butterfly2_0/twiddle/bus_mult/a_debus ==
  bus_in : Inport
  reinterpret1 : xbsIndex_r4/Reinterpret  force_arith_type=on  arith_type=Unsigned  force_bin_pt=on  bin_pt=0  block_type=reinterpret
  slice1 : xbsIndex_r4/Slice  nbits=36  boolean_output=off  mode=Upper Bit Location + Width  bit1=0  base1=MSB of Input  bit0=0  base0=LSB of Input  dbl_ovrd=off  block_type=slice
  msb_lsb_out1 : Outport
  wires:
  bus_in/1 -> slice1/1
  slice1/1 -> reinterpret1/1
  reinterpret1/1 -> msb_lsb_out1/1
